simulink model "dpsim_rlc_3ph_me"  (R2025a)
settings: Solver=ode45  StartTime=0  StopTime=0.10000000000000001  MaxStep=1.0000000000000001e-05  RelTol=1e-9  AbsTol=1e-10
settings Model: Creator=matthiasmees  LastModifiedBy=matthiasmees

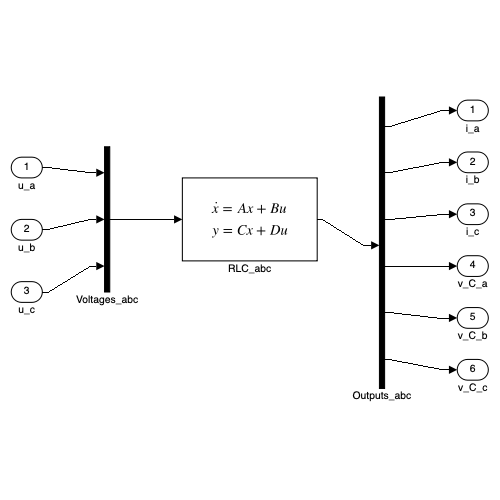
[thumbnail: Simulink's stored preview of the top-level diagram]
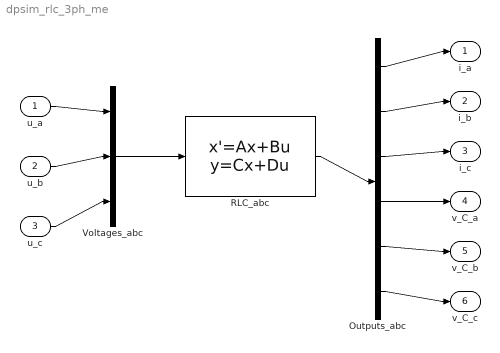
== system dpsim_rlc_3ph_me ==
  u_a : Inport  OutDataTypeStr=double  PortDimensions=1  SampleTime=0
  u_b : Inport  Port=2  OutDataTypeStr=double  PortDimensions=1  SampleTime=0
  u_c : Inport  Port=3  OutDataTypeStr=double  PortDimensions=1  SampleTime=0
  Outputs_abc : Demux  Outputs=6
  RLC_abc : StateSpace  A=[-500 0 0 -50 0 0;0 -500 0 0 -50 0;0 0 -500 0 0 -50;10000 0 0 0 0 0;0 10000 0 0 0 0;0 0 10000 0 0 0]  B=[50 0 0;0 50 0;0 0 50;0 0 0;0 0 0;0 0 0]  C=[1 0 0 0 0 0;0 1 0 0 0 0;0 0 1 0 0 0;0 0 0 1 0 0;0 0 0 0 1 0;0 0 0 0 0 1]  D=[0 0 0;0 0 0;0 0 0;0 0 0;0 0 0;0 0 0]  InitialCondition=[0;0;0;0;0;0]
  Voltages_abc : Mux  Inputs=3
  i_a : Outport
  i_b : Outport  Port=2
  i_c : Outport  Port=3
  v_C_a : Outport  Port=4
  v_C_b : Outport  Port=5
  v_C_c : Outport  Port=6
  wires:
  u_a/1 -> Voltages_abc/1
  u_b/1 -> Voltages_abc/2
  u_c/1 -> Voltages_abc/3
  Voltages_abc/1 -> RLC_abc/1
  RLC_abc/1 -> Outputs_abc/1
  Outputs_abc/1 -> i_a/1
  Outputs_abc/2 -> i_b/1
  Outputs_abc/3 -> i_c/1
  Outputs_abc/4 -> v_C_a/1
  Outputs_abc/5 -> v_C_b/1
  Outputs_abc/6 -> v_C_c/1
